simulink model "afe_dq_ttype"  (R2026b)
settings: Solver=ode23tb  StopTime=param.sim.simlength  FixedStep=param.sim.tc  MaxStep=param.glb_time.tc
values from neighbouring files (symbols this model uses):
  param = struct()    [init_model.m]
undefined symbols (not defined in the file or in its folder): magnitude
libraries: fl_lib x281, nesl_utility x136, igbt_simple_2th_lib x12, single_phase_transformer_lib x3, discrete_time_low_pass_filter x1, threephase_inductor_lib x1, dclink_for_three_levels x1, three_phase_three_level_ttype_inverter_ideal_switch_based_model x1, three_phase_three_levels_PWM_modulator x1, three_phase_bridge_three_level_ttype_igbt_simple_2th x1, three_phase_voltage_with_frt_emulator_mfcn x1
(part 3 of 8)

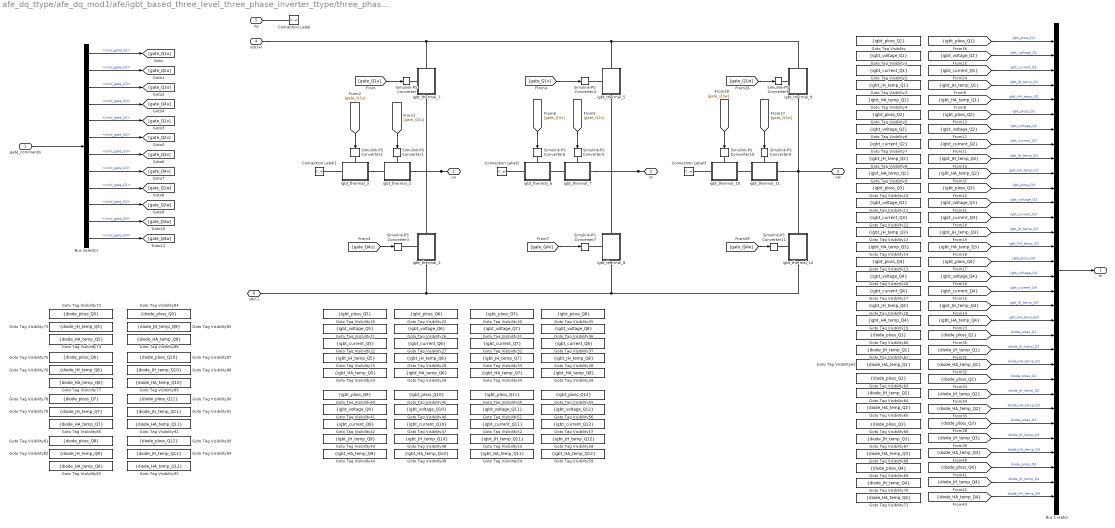
== system afe_dq_ttype/afe_dq_mod1/afe/igbt_based_three_level_three_phase_inverter_ttype/three_phase_inverter_igbt_2th_based_ttype ==
  gate_commands : Inport
  Bus Creator : BusCreator  Inputs=32
  Bus Selector : BusSelector  OutputSignals=gate_cmds_phu.cmd_gate_Q1,gate_cmds_phu.cmd_gate_Q2,gate_cmds_phu.cmd_gate_Q3,gate_cmds_phu.cmd_gate_Q4,gate_cmds_phv.cmd_gate_Q1,gate_cmds_phv.cmd_gate_Q2,gate_cmds_phv.cmd_gate_Q3,gate_cmds_phv.cmd_gate_Q4,gate_cmds_phw.cmd_gate_Q1,gate_cmds_phw.cmd_gate_Q2,gate_cmds_phw.cmd_gate_Q3,gate_cmds_phw.cmd_gate_Q4
  Connection Label{,1..3} (4 alike) : ConnectionLabel  Label=np
  Goto Tag Visibility : GotoTagVisibility  GotoTag=igbt_ploss_Q1
  Goto Tag Visibility1 : GotoTagVisibility  GotoTag=igbt_voltage_Q1
  Goto Tag Visibility10 : GotoTagVisibility  GotoTag=igbt_ploss_Q3
  Goto Tag Visibility11 : GotoTagVisibility  GotoTag=igbt_voltage_Q3
  Goto Tag Visibility12 : GotoTagVisibility  GotoTag=igbt_current_Q3
  Goto Tag Visibility13 : GotoTagVisibility  GotoTag=igbt_JH_temp_Q3
  Goto Tag Visibility14 : GotoTagVisibility  GotoTag=igbt_HA_temp_Q3
  Goto Tag Visibility15 : GotoTagVisibility  GotoTag=igbt_ploss_Q4
  Goto Tag Visibility16 : GotoTagVisibility  GotoTag=igbt_voltage_Q4
  Goto Tag Visibility17 : GotoTagVisibility  GotoTag=igbt_current_Q4
  Goto Tag Visibility18 : GotoTagVisibility  GotoTag=igbt_JH_temp_Q4
  Goto Tag Visibility19 : GotoTagVisibility  GotoTag=igbt_HA_temp_Q4
  Goto Tag Visibility2 : GotoTagVisibility  GotoTag=igbt_current_Q1
  Goto Tag Visibility20 : GotoTagVisibility  GotoTag=igbt_ploss_Q5
  Goto Tag Visibility21 : GotoTagVisibility  GotoTag=igbt_voltage_Q5
  Goto Tag Visibility22 : GotoTagVisibility  GotoTag=igbt_current_Q5
  Goto Tag Visibility23 : GotoTagVisibility  GotoTag=igbt_JH_temp_Q5
  Goto Tag Visibility24 : GotoTagVisibility  GotoTag=igbt_HA_temp_Q5
  Goto Tag Visibility25 : GotoTagVisibility  GotoTag=igbt_ploss_Q6
  Goto Tag Visibility26 : GotoTagVisibility  GotoTag=igbt_voltage_Q6
  Goto Tag Visibility27 : GotoTagVisibility  GotoTag=igbt_current_Q6
  Goto Tag Visibility28 : GotoTagVisibility  GotoTag=igbt_JH_temp_Q6
  Goto Tag Visibility29 : GotoTagVisibility  GotoTag=igbt_HA_temp_Q6
  Goto Tag Visibility3 : GotoTagVisibility  GotoTag=igbt_JH_temp_Q1
  Goto Tag Visibility30 : GotoTagVisibility  GotoTag=igbt_ploss_Q7
  Goto Tag Visibility31 : GotoTagVisibility  GotoTag=igbt_voltage_Q7
  Goto Tag Visibility32 : GotoTagVisibility  GotoTag=igbt_current_Q7
  Goto Tag Visibility33 : GotoTagVisibility  GotoTag=igbt_JH_temp_Q7
  Goto Tag Visibility34 : GotoTagVisibility  GotoTag=igbt_HA_temp_Q7
  Goto Tag Visibility35 : GotoTagVisibility  GotoTag=igbt_ploss_Q8
  Goto Tag Visibility36 : GotoTagVisibility  GotoTag=igbt_voltage_Q8
  Goto Tag Visibility37 : GotoTagVisibility  GotoTag=igbt_current_Q8
  Goto Tag Visibility38 : GotoTagVisibility  GotoTag=igbt_JH_temp_Q8
  Goto Tag Visibility39 : GotoTagVisibility  GotoTag=igbt_HA_temp_Q8
  Goto Tag Visibility4 : GotoTagVisibility  GotoTag=igbt_HA_temp_Q1
  Goto Tag Visibility40 : GotoTagVisibility  GotoTag=igbt_ploss_Q9
  Goto Tag Visibility41 : GotoTagVisibility  GotoTag=igbt_voltage_Q9
  Goto Tag Visibility42 : GotoTagVisibility  GotoTag=igbt_current_Q9
  Goto Tag Visibility43 : GotoTagVisibility  GotoTag=igbt_JH_temp_Q9
  Goto Tag Visibility44 : GotoTagVisibility  GotoTag=igbt_HA_temp_Q9
  Goto Tag Visibility45 : GotoTagVisibility  GotoTag=igbt_ploss_Q10
  Goto Tag Visibility46 : GotoTagVisibility  GotoTag=igbt_voltage_Q10
  Goto Tag Visibility47 : GotoTagVisibility  GotoTag=igbt_current_Q10
  Goto Tag Visibility48 : GotoTagVisibility  GotoTag=igbt_JH_temp_Q10
  Goto Tag Visibility49 : GotoTagVisibility  GotoTag=igbt_HA_temp_Q10
  Goto Tag Visibility5 : GotoTagVisibility  GotoTag=igbt_ploss_Q2
  Goto Tag Visibility50 : GotoTagVisibility  GotoTag=igbt_ploss_Q11
  Goto Tag Visibility51 : GotoTagVisibility  GotoTag=igbt_voltage_Q11
  Goto Tag Visibility52 : GotoTagVisibility  GotoTag=igbt_current_Q11
  Goto Tag Visibility53 : GotoTagVisibility  GotoTag=igbt_JH_temp_Q11
  Goto Tag Visibility54 : GotoTagVisibility  GotoTag=igbt_HA_temp_Q11
  Goto Tag Visibility55 : GotoTagVisibility  GotoTag=igbt_ploss_Q12
  Goto Tag Visibility56 : GotoTagVisibility  GotoTag=igbt_voltage_Q12
  Goto Tag Visibility57 : GotoTagVisibility  GotoTag=igbt_current_Q12
  Goto Tag Visibility58 : GotoTagVisibility  GotoTag=igbt_JH_temp_Q12
  Goto Tag Visibility59 : GotoTagVisibility  GotoTag=igbt_HA_temp_Q12
  Goto Tag Visibility6 : GotoTagVisibility  GotoTag=igbt_voltage_Q2
  Goto Tag Visibility60 : GotoTagVisibility  GotoTag=diode_ploss_Q1
  Goto Tag Visibility61 : GotoTagVisibility  GotoTag=diode_JH_temp_Q1
  Goto Tag Visibility62 : GotoTagVisibility  GotoTag=diode_HA_temp_Q1
  Goto Tag Visibility63 : GotoTagVisibility  GotoTag=diode_ploss_Q2
  Goto Tag Visibility64 : GotoTagVisibility  GotoTag=diode_JH_temp_Q2
  Goto Tag Visibility65 : GotoTagVisibility  GotoTag=diode_HA_temp_Q2
  Goto Tag Visibility66 : GotoTagVisibility  GotoTag=diode_ploss_Q3
  Goto Tag Visibility67 : GotoTagVisibility  GotoTag=diode_JH_temp_Q3
  Goto Tag Visibility68 : GotoTagVisibility  GotoTag=diode_HA_temp_Q3
  Goto Tag Visibility69 : GotoTagVisibility  GotoTag=diode_ploss_Q4
  Goto Tag Visibility7 : GotoTagVisibility  GotoTag=igbt_current_Q2
  Goto Tag Visibility70 : GotoTagVisibility  GotoTag=diode_JH_temp_Q4
  Goto Tag Visibility71 : GotoTagVisibility  GotoTag=diode_HA_temp_Q4
  Goto Tag Visibility72 : GotoTagVisibility  GotoTag=diode_ploss_Q5
  Goto Tag Visibility73 : GotoTagVisibility  GotoTag=diode_JH_temp_Q5
  Goto Tag Visibility74 : GotoTagVisibility  GotoTag=diode_HA_temp_Q5
  Goto Tag Visibility75 : GotoTagVisibility  GotoTag=diode_ploss_Q6
  Goto Tag Visibility76 : GotoTagVisibility  GotoTag=diode_JH_temp_Q6
  Goto Tag Visibility77 : GotoTagVisibility  GotoTag=diode_HA_temp_Q6
  Goto Tag Visibility78 : GotoTagVisibility  GotoTag=diode_ploss_Q7
  Goto Tag Visibility79 : GotoTagVisibility  GotoTag=diode_JH_temp_Q7
  Goto Tag Visibility8 : GotoTagVisibility  GotoTag=igbt_JH_temp_Q2
  Goto Tag Visibility80 : GotoTagVisibility  GotoTag=diode_HA_temp_Q7
  Goto Tag Visibility81 : GotoTagVisibility  GotoTag=diode_ploss_Q8
  Goto Tag Visibility82 : GotoTagVisibility  GotoTag=diode_JH_temp_Q8
  Goto Tag Visibility83 : GotoTagVisibility  GotoTag=diode_HA_temp_Q8
  Goto Tag Visibility84 : GotoTagVisibility  GotoTag=diode_ploss_Q9
  Goto Tag Visibility85 : GotoTagVisibility  GotoTag=diode_JH_temp_Q9
  Goto Tag Visibility86 : GotoTagVisibility  GotoTag=diode_HA_temp_Q9
  Goto Tag Visibility87 : GotoTagVisibility  GotoTag=diode_ploss_Q10
  Goto Tag Visibility88 : GotoTagVisibility  GotoTag=diode_JH_temp_Q10
  Goto Tag Visibility89 : GotoTagVisibility  GotoTag=diode_HA_temp_Q10
  Goto Tag Visibility9 : GotoTagVisibility  GotoTag=igbt_HA_temp_Q2
  Goto Tag Visibility90 : GotoTagVisibility  GotoTag=diode_ploss_Q11
  Goto Tag Visibility91 : GotoTagVisibility  GotoTag=diode_JH_temp_Q11
  Goto Tag Visibility92 : GotoTagVisibility  GotoTag=diode_HA_temp_Q11
  Goto Tag Visibility93 : GotoTagVisibility  GotoTag=diode_ploss_Q12
  Goto Tag Visibility94 : GotoTagVisibility  GotoTag=diode_JH_temp_Q12
  Goto Tag Visibility95 : GotoTagVisibility  GotoTag=diode_HA_temp_Q12
  Simulink-PS Converter{,1..11} (12 alike) : nesl_utility/Simulink-PS Converter  PhysicalDomain=network_engine_domain  SubClassName=ps_input  LeftPortType=input  RightPortType=output  PseudoPeriodic=off  Frequencies=[]  NoiseDistribution=none  NoiseParameters=[]  Unit=1  AffineConversion=on  FilteringAndDerivatives=provide  SimscapeFilterOrder=1  InputFilterTimeConstant=0.001  UdotUserProvided=0
  igbt_thermal_1 : Subsystem
      settings: PortSchema="{\"entries\":[{\"content\":{\"sides\":[{\"content\":{\"connectorIds\":[\"LConn1\"]},\"type\":\"ConnectorPlacement.EquallySpacedRectSide\",\"uuid\":\"9277da8d-d460-43e6-8478-dd662f15d226\"},{\"content\":{\"connectorIds\":[],\"side\":\"RIGHT\"},\"type\":\"ConnectorPlacement.EquallySpacedRectSide\",\"uuid\":\"a7ece396-f1d9-4f4f-a05b-db1fc65d6e1d\"},{\"content\":{\"connectorIds\":[\"LConn2\"],\"side\":\"TOP\"},\"type\":\"ConnectorPlacement.EquallySpacedRectSide\",\"uuid\":\"fdd70777-e9cf-4317-afb6-cae87f75d5b0\"},{\"content\":{\"connectorIds\":[\"RConn1\"],\"side\":\"BOTTOM\"},\"type\":\"ConnectorPlacement.EquallySpacedRectSide\",\"uuid\":\"2353ed68-b1a1-4775-9ca9-31e268d5443b\"}]},\"type\":\"ConnectorPlacement.EquallySpacedConnector\",\"uuid\":\"d5479f4c-4e65-4791-adcb-73df11f88590\"}],\"packageUris\":[\"http://schema.mathworks.com/mf0/Connector/R2020b\"],\"version\":\"1.0\"}"
  igbt_thermal_10 : Subsystem
      settings: PortSchema="{\"entries\":[{\"content\":{\"sides\":[{\"content\":{\"connectorIds\":[\"LConn1\"]},\"type\":\"ConnectorPlacement.EquallySpacedRectSide\",\"uuid\":\"9277da8d-d460-43e6-8478-dd662f15d226\"},{\"content\":{\"connectorIds\":[],\"side\":\"RIGHT\"},\"type\":\"ConnectorPlacement.EquallySpacedRectSide\",\"uuid\":\"a7ece396-f1d9-4f4f-a05b-db1fc65d6e1d\"},{\"content\":{\"connectorIds\":[\"LConn2\"],\"side\":\"TOP\"},\"type\":\"ConnectorPlacement.EquallySpacedRectSide\",\"uuid\":\"fdd70777-e9cf-4317-afb6-cae87f75d5b0\"},{\"content\":{\"connectorIds\":[\"RConn1\"],\"side\":\"BOTTOM\"},\"type\":\"ConnectorPlacement.EquallySpacedRectSide\",\"uuid\":\"2353ed68-b1a1-4775-9ca9-31e268d5443b\"}]},\"type\":\"ConnectorPlacement.EquallySpacedConnector\",\"uuid\":\"d5479f4c-4e65-4791-adcb-73df11f88590\"}],\"packageUris\":[\"http://schema.mathworks.com/mf0/Connector/R2020b\"],\"version\":\"1.0\"}"
  igbt_thermal_11 : Subsystem
      settings: PortSchema="{\"entries\":[{\"content\":{\"sides\":[{\"content\":{\"connectorIds\":[\"LConn1\"]},\"type\":\"ConnectorPlacement.EquallySpacedRectSide\",\"uuid\":\"9277da8d-d460-43e6-8478-dd662f15d226\"},{\"content\":{\"connectorIds\":[],\"side\":\"RIGHT\"},\"type\":\"ConnectorPlacement.EquallySpacedRectSide\",\"uuid\":\"a7ece396-f1d9-4f4f-a05b-db1fc65d6e1d\"},{\"content\":{\"connectorIds\":[\"LConn2\"],\"side\":\"TOP\"},\"type\":\"ConnectorPlacement.EquallySpacedRectSide\",\"uuid\":\"fdd70777-e9cf-4317-afb6-cae87f75d5b0\"},{\"content\":{\"connectorIds\":[\"RConn1\"],\"side\":\"BOTTOM\"},\"type\":\"ConnectorPlacement.EquallySpacedRectSide\",\"uuid\":\"2353ed68-b1a1-4775-9ca9-31e268d5443b\"}]},\"type\":\"ConnectorPlacement.EquallySpacedConnector\",\"uuid\":\"d5479f4c-4e65-4791-adcb-73df11f88590\"}],\"packageUris\":[\"http://schema.mathworks.com/mf0/Connector/R2020b\"],\"version\":\"1.0\"}"
  igbt_thermal_12 : Subsystem
      settings: PortSchema="{\"entries\":[{\"content\":{\"sides\":[{\"content\":{\"connectorIds\":[\"LConn1\"]},\"type\":\"ConnectorPlacement.EquallySpacedRectSide\",\"uuid\":\"9277da8d-d460-43e6-8478-dd662f15d226\"},{\"content\":{\"connectorIds\":[],\"side\":\"RIGHT\"},\"type\":\"ConnectorPlacement.EquallySpacedRectSide\",\"uuid\":\"a7ece396-f1d9-4f4f-a05b-db1fc65d6e1d\"},{\"content\":{\"connectorIds\":[\"LConn2\"],\"side\":\"TOP\"},\"type\":\"ConnectorPlacement.EquallySpacedRectSide\",\"uuid\":\"fdd70777-e9cf-4317-afb6-cae87f75d5b0\"},{\"content\":{\"connectorIds\":[\"RConn1\"],\"side\":\"BOTTOM\"},\"type\":\"ConnectorPlacement.EquallySpacedRectSide\",\"uuid\":\"2353ed68-b1a1-4775-9ca9-31e268d5443b\"}]},\"type\":\"ConnectorPlacement.EquallySpacedConnector\",\"uuid\":\"d5479f4c-4e65-4791-adcb-73df11f88590\"}],\"packageUris\":[\"http://schema.mathworks.com/mf0/Connector/R2020b\"],\"version\":\"1.0\"}"
  igbt_thermal_2 : Subsystem
      settings: PortSchema="{\"entries\":[{\"content\":{\"sides\":[{\"content\":{\"connectorIds\":[\"LConn1\"]},\"type\":\"ConnectorPlacement.EquallySpacedRectSide\",\"uuid\":\"9277da8d-d460-43e6-8478-dd662f15d226\"},{\"content\":{\"connectorIds\":[],\"side\":\"RIGHT\"},\"type\":\"ConnectorPlacement.EquallySpacedRectSide\",\"uuid\":\"a7ece396-f1d9-4f4f-a05b-db1fc65d6e1d\"},{\"content\":{\"connectorIds\":[\"LConn2\"],\"side\":\"TOP\"},\"type\":\"ConnectorPlacement.EquallySpacedRectSide\",\"uuid\":\"fdd70777-e9cf-4317-afb6-cae87f75d5b0\"},{\"content\":{\"connectorIds\":[\"RConn1\"],\"side\":\"BOTTOM\"},\"type\":\"ConnectorPlacement.EquallySpacedRectSide\",\"uuid\":\"2353ed68-b1a1-4775-9ca9-31e268d5443b\"}]},\"type\":\"ConnectorPlacement.EquallySpacedConnector\",\"uuid\":\"d5479f4c-4e65-4791-adcb-73df11f88590\"}],\"packageUris\":[\"http://schema.mathworks.com/mf0/Connector/R2020b\"],\"version\":\"1.0\"}"
  igbt_thermal_3 : Subsystem
      settings: PortSchema="{\"entries\":[{\"content\":{\"sides\":[{\"content\":{\"connectorIds\":[\"LConn1\"]},\"type\":\"ConnectorPlacement.EquallySpacedRectSide\",\"uuid\":\"9277da8d-d460-43e6-8478-dd662f15d226\"},{\"content\":{\"side\":\"RIGHT\"},\"type\":\"ConnectorPlacement.EquallySpacedRectSide\",\"uuid\":\"a7ece396-f1d9-4f4f-a05b-db1fc65d6e1d\"},{\"content\":{\"connectorIds\":[\"LConn2\"],\"side\":\"TOP\"},\"type\":\"ConnectorPlacement.EquallySpacedRectSide\",\"uuid\":\"fdd70777-e9cf-4317-afb6-cae87f75d5b0\"},{\"content\":{\"connectorIds\":[\"RConn1\"],\"side\":\"BOTTOM\"},\"type\":\"ConnectorPlacement.EquallySpacedRectSide\",\"uuid\":\"2353ed68-b1a1-4775-9ca9-31e268d5443b\"}]},\"type\":\"ConnectorPlacement.EquallySpacedConnector\",\"uuid\":\"d5479f4c-4e65-4791-adcb-73df11f88590\"}],\"packageUris\":[\"http://schema.mathworks.com/mf0/Connector/R2020b\"],\"version\":\"1.0\"}"
  igbt_thermal_4 : Subsystem
      settings: PortSchema="{\"entries\":[{\"content\":{\"sides\":[{\"content\":{\"connectorIds\":[\"LConn1\"]},\"type\":\"ConnectorPlacement.EquallySpacedRectSide\",\"uuid\":\"9277da8d-d460-43e6-8478-dd662f15d226\"},{\"content\":{\"connectorIds\":[],\"side\":\"RIGHT\"},\"type\":\"ConnectorPlacement.EquallySpacedRectSide\",\"uuid\":\"a7ece396-f1d9-4f4f-a05b-db1fc65d6e1d\"},{\"content\":{\"connectorIds\":[\"LConn2\"],\"side\":\"TOP\"},\"type\":\"ConnectorPlacement.EquallySpacedRectSide\",\"uuid\":\"fdd70777-e9cf-4317-afb6-cae87f75d5b0\"},{\"content\":{\"connectorIds\":[\"RConn1\"],\"side\":\"BOTTOM\"},\"type\":\"ConnectorPlacement.EquallySpacedRectSide\",\"uuid\":\"2353ed68-b1a1-4775-9ca9-31e268d5443b\"}]},\"type\":\"ConnectorPlacement.EquallySpacedConnector\",\"uuid\":\"d5479f4c-4e65-4791-adcb-73df11f88590\"}],\"packageUris\":[\"http://schema.mathworks.com/mf0/Connector/R2020b\"],\"version\":\"1.0\"}"
  igbt_thermal_5 : Subsystem
      settings: PortSchema="{\"entries\":[{\"content\":{\"sides\":[{\"content\":{\"connectorIds\":[\"LConn1\"]},\"type\":\"ConnectorPlacement.EquallySpacedRectSide\",\"uuid\":\"9277da8d-d460-43e6-8478-dd662f15d226\"},{\"content\":{\"connectorIds\":[],\"side\":\"RIGHT\"},\"type\":\"ConnectorPlacement.EquallySpacedRectSide\",\"uuid\":\"a7ece396-f1d9-4f4f-a05b-db1fc65d6e1d\"},{\"content\":{\"connectorIds\":[\"LConn2\"],\"side\":\"TOP\"},\"type\":\"ConnectorPlacement.EquallySpacedRectSide\",\"uuid\":\"fdd70777-e9cf-4317-afb6-cae87f75d5b0\"},{\"content\":{\"connectorIds\":[\"RConn1\"],\"side\":\"BOTTOM\"},\"type\":\"ConnectorPlacement.EquallySpacedRectSide\",\"uuid\":\"2353ed68-b1a1-4775-9ca9-31e268d5443b\"}]},\"type\":\"ConnectorPlacement.EquallySpacedConnector\",\"uuid\":\"d5479f4c-4e65-4791-adcb-73df11f88590\"}],\"packageUris\":[\"http://schema.mathworks.com/mf0/Connector/R2020b\"],\"version\":\"1.0\"}"
  igbt_thermal_6 : Subsystem
      settings: PortSchema="{\"entries\":[{\"content\":{\"sides\":[{\"content\":{\"connectorIds\":[\"LConn1\"]},\"type\":\"ConnectorPlacement.EquallySpacedRectSide\",\"uuid\":\"9277da8d-d460-43e6-8478-dd662f15d226\"},{\"content\":{\"side\":\"RIGHT\"},\"type\":\"ConnectorPlacement.EquallySpacedRectSide\",\"uuid\":\"a7ece396-f1d9-4f4f-a05b-db1fc65d6e1d\"},{\"content\":{\"connectorIds\":[\"LConn2\"],\"side\":\"TOP\"},\"type\":\"ConnectorPlacement.EquallySpacedRectSide\",\"uuid\":\"fdd70777-e9cf-4317-afb6-cae87f75d5b0\"},{\"content\":{\"connectorIds\":[\"RConn1\"],\"side\":\"BOTTOM\"},\"type\":\"ConnectorPlacement.EquallySpacedRectSide\",\"uuid\":\"2353ed68-b1a1-4775-9ca9-31e268d5443b\"}]},\"type\":\"ConnectorPlacement.EquallySpacedConnector\",\"uuid\":\"d5479f4c-4e65-4791-adcb-73df11f88590\"}],\"packageUris\":[\"http://schema.mathworks.com/mf0/Connector/R2020b\"],\"version\":\"1.0\"}"
  igbt_thermal_7 : Subsystem
      settings: PortSchema="{\"entries\":[{\"content\":{\"sides\":[{\"content\":{\"connectorIds\":[\"LConn1\"]},\"type\":\"ConnectorPlacement.EquallySpacedRectSide\",\"uuid\":\"9277da8d-d460-43e6-8478-dd662f15d226\"},{\"content\":{\"connectorIds\":[],\"side\":\"RIGHT\"},\"type\":\"ConnectorPlacement.EquallySpacedRectSide\",\"uuid\":\"a7ece396-f1d9-4f4f-a05b-db1fc65d6e1d\"},{\"content\":{\"connectorIds\":[\"LConn2\"],\"side\":\"TOP\"},\"type\":\"ConnectorPlacement.EquallySpacedRectSide\",\"uuid\":\"fdd70777-e9cf-4317-afb6-cae87f75d5b0\"},{\"content\":{\"connectorIds\":[\"RConn1\"],\"side\":\"BOTTOM\"},\"type\":\"ConnectorPlacement.EquallySpacedRectSide\",\"uuid\":\"2353ed68-b1a1-4775-9ca9-31e268d5443b\"}]},\"type\":\"ConnectorPlacement.EquallySpacedConnector\",\"uuid\":\"d5479f4c-4e65-4791-adcb-73df11f88590\"}],\"packageUris\":[\"http://schema.mathworks.com/mf0/Connector/R2020b\"],\"version\":\"1.0\"}"
  igbt_thermal_8 : Subsystem
      settings: PortSchema="{\"entries\":[{\"content\":{\"sides\":[{\"content\":{\"connectorIds\":[\"LConn1\"]},\"type\":\"ConnectorPlacement.EquallySpacedRectSide\",\"uuid\":\"9277da8d-d460-43e6-8478-dd662f15d226\"},{\"content\":{\"connectorIds\":[],\"side\":\"RIGHT\"},\"type\":\"ConnectorPlacement.EquallySpacedRectSide\",\"uuid\":\"a7ece396-f1d9-4f4f-a05b-db1fc65d6e1d\"},{\"content\":{\"connectorIds\":[\"LConn2\"],\"side\":\"TOP\"},\"type\":\"ConnectorPlacement.EquallySpacedRectSide\",\"uuid\":\"fdd70777-e9cf-4317-afb6-cae87f75d5b0\"},{\"content\":{\"connectorIds\":[\"RConn1\"],\"side\":\"BOTTOM\"},\"type\":\"ConnectorPlacement.EquallySpacedRectSide\",\"uuid\":\"2353ed68-b1a1-4775-9ca9-31e268d5443b\"}]},\"type\":\"ConnectorPlacement.EquallySpacedConnector\",\"uuid\":\"d5479f4c-4e65-4791-adcb-73df11f88590\"}],\"packageUris\":[\"http://schema.mathworks.com/mf0/Connector/R2020b\"],\"version\":\"1.0\"}"
  igbt_thermal_9 : Subsystem
      settings: PortSchema="{\"entries\":[{\"content\":{\"sides\":[{\"content\":{\"connectorIds\":[\"LConn1\"]},\"type\":\"ConnectorPlacement.EquallySpacedRectSide\",\"uuid\":\"9277da8d-d460-43e6-8478-dd662f15d226\"},{\"content\":{\"connectorIds\":[],\"side\":\"RIGHT\"},\"type\":\"ConnectorPlacement.EquallySpacedRectSide\",\"uuid\":\"a7ece396-f1d9-4f4f-a05b-db1fc65d6e1d\"},{\"content\":{\"connectorIds\":[\"LConn2\"],\"side\":\"TOP\"},\"type\":\"ConnectorPlacement.EquallySpacedRectSide\",\"uuid\":\"fdd70777-e9cf-4317-afb6-cae87f75d5b0\"},{\"content\":{\"connectorIds\":[\"RConn1\"],\"side\":\"BOTTOM\"},\"type\":\"ConnectorPlacement.EquallySpacedRectSide\",\"uuid\":\"2353ed68-b1a1-4775-9ca9-31e268d5443b\"}]},\"type\":\"ConnectorPlacement.EquallySpacedConnector\",\"uuid\":\"d5479f4c-4e65-4791-adcb-73df11f88590\"}],\"packageUris\":[\"http://schema.mathworks.com/mf0/Connector/R2020b\"],\"version\":\"1.0\"}"
  uu : PMIOPort  Side=Left
  uv : PMIOPort  Port=2  Side=Left
  uw : PMIOPort  Port=3  Side=Left
  udc(+) : PMIOPort  Port=4  Side=Right
  np : PMIOPort  Port=5  Side=Right
  udc(-) : PMIOPort  Port=6  Side=Right
  m : Outport
  wires:
  [gate_Q4u] -> Simulink-PS Converter3/1
  [gate_Q3u] -> Simulink-PS Converter2/1
  [gate_Q2u] -> Simulink-PS Converter1/1
  [gate_Q1u] -> Simulink-PS Converter/1
  [gate_Q1v] -> Simulink-PS Converter4/1
  [gate_Q2v] -> Simulink-PS Converter5/1
  [gate_Q3v] -> Simulink-PS Converter6/1
  [gate_Q4v] -> Simulink-PS Converter7/1
  gate_commands/1 -> Bus Selector/1
  [igbt_voltage_Q1] -> Bus Creator/2  "igbt_voltage_Q1"
  [igbt_current_Q4] -> Bus Creator/18  "igbt_current_Q4"
  [igbt_voltage_Q2] -> Bus Creator/7  "igbt_voltage_Q2"
  [igbt_ploss_Q2] -> Bus Creator/6  "igbt_ploss_Q2"
  Bus Creator/1 -> m/1
  [igbt_ploss_Q3] -> Bus Creator/11  "igbt_ploss_Q3"
  [igbt_HA_temp_Q1] -> Bus Creator/5  "igbt_HA_temp_Q1"
  [igbt_ploss_Q1] -> Bus Creator/1  "igbt_ploss_Q1"
  [igbt_voltage_Q4] -> Bus Creator/17  "igbt_voltage_Q4"
  [igbt_ploss_Q4] -> Bus Creator/16  "igbt_ploss_Q4"
  [igbt_JH_temp_Q4] -> Bus Creator/19  "igbt_JH_temp_Q4"
  [igbt_voltage_Q3] -> Bus Creator/12  "igbt_voltage_Q3"
  [igbt_current_Q1] -> Bus Creator/3  "igbt_current_Q1"
  [igbt_HA_temp_Q4] -> Bus Creator/20  "igbt_HA_temp_Q4"
  [igbt_JH_temp_Q3] -> Bus Creator/14  "igbt_JH_temp_Q3"
  [igbt_current_Q2] -> Bus Creator/8  "igbt_current_Q2"
  [igbt_HA_temp_Q2] -> Bus Creator/10  "igbt_HA_temp_Q2"
  [igbt_JH_temp_Q2] -> Bus Creator/9  "igbt_JH_temp_Q2"
  [igbt_JH_temp_Q1] -> Bus Creator/4  "igbt_JH_temp_Q1"
  [igbt_current_Q3] -> Bus Creator/13  "igbt_current_Q3"
  [igbt_HA_temp_Q3] -> Bus Creator/15  "igbt_HA_temp_Q3"
  [gate_Q4w] -> Simulink-PS Converter11/1
  [gate_Q3w] -> Simulink-PS Converter10/1
  [gate_Q2w] -> Simulink-PS Converter9/1
  [gate_Q1w] -> Simulink-PS Converter8/1
  [diode_ploss_Q1] -> Bus Creator/21  "diode_ploss_Q1"
  [diode_JH_temp_Q1] -> Bus Creator/22  "diode_JH_temp_Q1"
  [diode_HA_temp_Q1] -> Bus Creator/23  "diode_HA_temp_Q1"
  [diode_ploss_Q2] -> Bus Creator/24  "diode_ploss_Q2"
  [diode_JH_temp_Q2] -> Bus Creator/25  "diode_JH_temp_Q2"
  [diode_HA_temp_Q2] -> Bus Creator/26  "diode_HA_temp_Q2"
  [diode_ploss_Q3] -> Bus Creator/27  "diode_ploss_Q3"
  [diode_JH_temp_Q3] -> Bus Creator/28  "diode_JH_temp_Q3"
  [diode_HA_temp_Q3] -> Bus Creator/29  "diode_HA_temp_Q3"
  [diode_HA_temp_Q4] -> Bus Creator/32  "diode_HA_temp_Q4"
  [diode_JH_temp_Q4] -> Bus Creator/31  "diode_JH_temp_Q4"
  [diode_ploss_Q4] -> Bus Creator/30  "diode_ploss_Q4"
  Bus Selector/1 -> [gate_Q1u]  "<cmd_gate_Q1>"
  Bus Selector/2 -> [gate_Q2u]  "<cmd_gate_Q2>"
  Bus Selector/3 -> [gate_Q3u]  "<cmd_gate_Q3>"
  Bus Selector/9 -> [gate_Q1w]  "<cmd_gate_Q1>"
  Bus Selector/4 -> [gate_Q4u]  "<cmd_gate_Q4>"
  Bus Selector/5 -> [gate_Q1v]  "<cmd_gate_Q1>"
  Bus Selector/6 -> [gate_Q2v]  "<cmd_gate_Q2>"
  Bus Selector/7 -> [gate_Q3v]  "<cmd_gate_Q3>"
  Bus Selector/8 -> [gate_Q4v]  "<cmd_gate_Q4>"
  Bus Selector/10 -> [gate_Q2w]  "<cmd_gate_Q2>"
  Bus Selector/12 -> [gate_Q4w]  "<cmd_gate_Q4>"
  Bus Selector/11 -> [gate_Q3w]  "<cmd_gate_Q3>"
  connections:
  udc(+)/RConn1 -- igbt_thermal_1/LConn2 -- igbt_thermal_5/LConn2 -- igbt_thermal_9/LConn2
  igbt_thermal_4/LConn1 -- Simulink-PS Converter3/RConn1
  igbt_thermal_3/LConn1 -- Simulink-PS Converter2/RConn1
  igbt_thermal_2/LConn1 -- Simulink-PS Converter1/RConn1
  igbt_thermal_1/LConn1 -- Simulink-PS Converter/RConn1
  igbt_thermal_7/LConn1 -- Simulink-PS Converter5/RConn1
  igbt_thermal_6/LConn1 -- Simulink-PS Converter6/RConn1
  igbt_thermal_8/LConn1 -- Simulink-PS Converter7/RConn1
  uu/RConn1 -- igbt_thermal_2/RConn1 -- igbt_thermal_4/LConn2 -- igbt_thermal_1/RConn1
  igbt_thermal_12/RConn1 -- igbt_thermal_8/RConn1 -- udc(-)/RConn1 -- igbt_thermal_4/RConn1
  uv/RConn1 -- igbt_thermal_5/RConn1 -- igbt_thermal_8/LConn2 -- igbt_thermal_7/RConn1
  igbt_thermal_7/LConn2 -- igbt_thermal_6/LConn2
  Connection Label/LConn1 -- np/RConn1
  igbt_thermal_3/RConn1 -- Connection Label1/LConn1
  igbt_thermal_6/RConn1 -- Connection Label2/LConn1
  igbt_thermal_9/RConn1 -- igbt_thermal_12/LConn2 -- igbt_thermal_11/RConn1 -- uw/RConn1
  igbt_thermal_9/LConn1 -- Simulink-PS Converter8/RConn1
  igbt_thermal_3/LConn2 -- igbt_thermal_2/LConn2
  igbt_thermal_12/LConn1 -- Simulink-PS Converter11/RConn1
  igbt_thermal_10/LConn1 -- Simulink-PS Converter10/RConn1
  igbt_thermal_10/RConn1 -- Connection Label3/LConn1
  igbt_thermal_11/LConn1 -- Simulink-PS Converter9/RConn1
  igbt_thermal_11/LConn2 -- igbt_thermal_10/LConn2
  igbt_thermal_5/LConn1 -- Simulink-PS Converter4/RConn1

== system afe_dq_ttype/afe_dq_mod1/afe/sv_pwm/modulator1 ==
  u : Inport
  v : Inport  Port=2
  w : Inport  Port=3
  phase : Inport  Port=4
  Bus Creator : BusCreator  Inputs=3
  three_phase_three_levels_PWM_generator_with_global_TRGO1 : three_phase_three_levels_PWM_modulator/three_phase_three_levels_PWM_generator_with_global_TRGO1  f=param.glb_time.fPWM_AFE  m_up=1  m_low=-1  dead_time=0  pos_cmd_gate=15  neg_cmd_gate=0  polarity=1  tc=param.glb_time.tc  double_sampling=param.glb_time.TRGO_AFE_double_update
      link override gate commands/Bus Selector: OutputSignals=du(t)
      link override gate commands/Bus Selector1: OutputSignals=dv(t)
      link override gate commands/Bus Selector2: OutputSignals=dw(t)
  gate_cmds : Outport
  tag scope: TRGO_afe_module_1=global
  wires:
  [time_afe_module_1] -> three_phase_three_levels_PWM_generator_with_global_TRGO1/1
  Bus Creator/1 -> three_phase_three_levels_PWM_generator_with_global_TRGO1/3
  three_phase_three_levels_PWM_generator_with_global_TRGO1/1 -> [TRGO_afe_module_1]
  u/1 -> Bus Creator/1  "du(t)"
  v/1 -> Bus Creator/2  "dv(t)"
  w/1 -> Bus Creator/3  "dw(t)"
  phase/1 -> three_phase_three_levels_PWM_generator_with_global_TRGO1/2
  three_phase_three_levels_PWM_generator_with_global_TRGO1/2 -> gate_cmds/1

== system afe_dq_ttype/afe_dq_mod1/AFE_control/afe_control/acquisitions/grid_phase_acquisition ==
  grid_phase : Inport
  Quantizer : Quantizer  QuantizationInterval=param.meas.adc_quantization
  Unit Delay : UnitDelay  SampleTime=-1
  Zero-Order Hold : ZeroOrderHold  SampleTime=-1
  grid_phased : Outport
  wires:
  Zero-Order Hold/1 -> Quantizer/1
  Unit Delay/1 -> grid_phased/1
  grid_phase/1 -> Zero-Order Hold/1
  Quantizer/1 -> Unit Delay/1

== system afe_dq_ttype/afe_dq_mod1/AFE_control/afe_control/acquisitions/ig afe quantizzation and one step delay ==
  ig_abc_pu : Inport
  Demux1 : Demux  Outputs=3
  Mux1 : Mux  Inputs=3
  ig afe quantizzation and one step delay : Subsystem
  igd_abc_pu : Outport
  wires:
  Demux1/1 -> ig afe quantizzation and one step delay/1(ig_u_pu)
  Demux1/2 -> ig afe quantizzation and one step delay/2(ig_v_pu)
  ig_abc_pu/1 -> Demux1/1
  Mux1/1 -> igd_abc_pu/1
  Demux1/3 -> ig afe quantizzation and one step delay/3(ig_w_pu)
  ig afe quantizzation and one step delay/2(igd_v_pu) -> Mux1/2
  ig afe quantizzation and one step delay/1(igd_u_pu) -> Mux1/1
  ig afe quantizzation and one step delay/3(igd_w_pu) -> Mux1/3

== system afe_dq_ttype/afe_dq_mod1/AFE_control/afe_control/acquisitions/is afe quantizzation and one step delay ==
  is_abc_pu : Inport
  Demux : Demux  Outputs=3
  Mux : Mux  Inputs=3
  is afe quantizzation and one step delay : Subsystem
  isd_abc_pu : Outport
  wires:
  is afe quantizzation and one step delay/2(isd_v_pu) -> Mux/2
  is_abc_pu/1 -> Demux/1
  is afe quantizzation and one step delay/3(isd_w_pu) -> Mux/3
  is afe quantizzation and one step delay/1(isd_u_pu) -> Mux/1
  Demux/1 -> is afe quantizzation and one step delay/1(is_u_pu)
  Mux/1 -> isd_abc_pu/1
  Demux/3 -> is afe quantizzation and one step delay/3(is_w_pu)
  Demux/2 -> is afe quantizzation and one step delay/2(is_v_pu)

== system afe_dq_ttype/afe_dq_mod1/AFE_control/afe_control/acquisitions/phase_compensation_1 ==
  local_time : Inport
  master_time : Inport  Port=2
  Zero-Order Hold : ZeroOrderHold  SampleTime=-1
  Zero-Order Hold1 : ZeroOrderHold  SampleTime=-1
  alignment_eval_afe1 : Subsystem
  y : Outport
  wires:
  local_time/1 -> Zero-Order Hold/1
  master_time/1 -> Zero-Order Hold1/1
  alignment_eval_afe1/1(dp) -> y/1
  Zero-Order Hold/1 -> alignment_eval_afe1/1(local_time)
  Zero-Order Hold1/1 -> alignment_eval_afe1/2(master_time)

== system afe_dq_ttype/afe_dq_mod1/AFE_control/afe_control/acquisitions/udc_acquisition ==
  udc_pu : Inport
  Quantizer : Quantizer  QuantizationInterval=param.meas.adc_quantization
  Unit Delay : UnitDelay  SampleTime=-1
  Zero-Order Hold : ZeroOrderHold  SampleTime=-1
  udcd_pu : Outport
  wires:
  Quantizer/1 -> Unit Delay/1
  udc_pu/1 -> Zero-Order Hold/1
  Unit Delay/1 -> udcd_pu/1
  Zero-Order Hold/1 -> Quantizer/1

== system afe_dq_ttype/afe_dq_mod1/AFE_control/afe_control/acquisitions/ug afe quantizzation and one step delay ==
  ug_abc_pu : Inport
  Demux : Demux  Outputs=3
  Mux : Mux  Inputs=3
  ug afe quantizzation and one step delay : Subsystem
  ugd_abc_pu : Outport
  wires:
  ug afe quantizzation and one step delay/2(ugd_v_pu) -> Mux/2
  Demux/2 -> ug afe quantizzation and one step delay/2(ug_v_pu)
  Demux/3 -> ug afe quantizzation and one step delay/3(ug_w_pu)
  ug afe quantizzation and one step delay/1(ugd_u_pu) -> Mux/1
  Demux/1 -> ug afe quantizzation and one step delay/1(ug_u_pu)
  ug_abc_pu/1 -> Demux/1
  ug afe quantizzation and one step delay/3(ugd_w_pu) -> Mux/3
  Mux/1 -> ugd_abc_pu/1

== system afe_dq_ttype/afe_dq_mod1/AFE_control/afe_control/current_ctrl/current_transformation ==
  is_a_pu : Inport
  is_b_pu : Inport  Port=2
  is_c_pu : Inport  Port=3
  alphabeta2xieta : MATLAB Function  TreatAsAtomicUnit=on
  uvw2alphabeta : MATLAB Function  TreatAsAtomicUnit=on
  tag scope: id_eta_pu=scoped, id_xi_pu=scoped
  wires:
  is_c_pu/1 -> uvw2alphabeta/3(w)
  alphabeta2xieta/2(eta) -> [id_eta_pu]  "ieta_pu"
  alphabeta2xieta/1(xi) -> [id_xi_pu]  "ixi_pu"
  is_b_pu/1 -> uvw2alphabeta/2(v)
  uvw2alphabeta/2(beta) -> alphabeta2xieta/2(beta)  "ibeta_pu"
  uvw2alphabeta/1(alpha) -> alphabeta2xieta/1(alpha)  "ialpha_pu"
  [phase_grid_pll] -> alphabeta2xieta/3(gamma)
  is_a_pu/1 -> uvw2alphabeta/1(u)

== system afe_dq_ttype/afe_dq_mod1/AFE_control/afe_control/current_ctrl/dq_vector_pi ==
  id : Inport
  id_ref : Inport  Port=2
  iq : Inport  Port=3
  iq_ref : Inport  Port=4
  Sum1 : Sum  Inputs=|-+
  Sum2 : Sum  Inputs=|-+
  bounder1 : Subsystem
  bounder2 : Subsystem
  pi_d : Subsystem
  pi_q : Subsystem
  switch : Subsystem
  vector lenght : Subsystem
  md_sat : Outport
  mq_sat : Outport  Port=2
  wires:
  bounder2/2(clip) -> switch/2(clip 2)
  vector lenght/2(m) -> bounder1/3(m), bounder2/1(m)
  Sum2/1 -> pi_q/1(iq_tilde)
  pi_d/1(ud_out) -> vector lenght/1(md), bounder1/1(md)
  pi_q/1(Vqs_out) -> bounder2/3(mq), vector lenght/2(mq)
  vector lenght/1(m_1) -> bounder1/2(m_1), bounder2/2(m_1)
  switch/1(clip) -> pi_q/2(clip), pi_d/2(clip)
  iq/1 -> Sum2/1
  Sum1/1 -> pi_d/1(id_tilde)
  bounder1/2(clip) -> switch/1(clip 1)
  id/1 -> Sum1/1
  bounder1/1(md_sat) -> md_sat/1
  bounder2/1(mq_sat) -> mq_sat/1
  id_ref/1 -> Sum1/2
  iq_ref/1 -> Sum2/2

== system afe_dq_ttype/afe_dq_mod1/AFE_control/afe_control/current_ctrl/zero_current_ctrl ==
  ualpha_ctrl_afe : Inport
  ubeta_ctrl_afe : Inport  Port=2
  Bus Creator1 : BusCreator  Inputs=3
  iz : Subsystem
  zero_sequence_current_ctrl : Subsystem
  uabg_ctrl_out : Outport
  wires:
  Bus Creator1/1 -> uabg_ctrl_out/1
  ualpha_ctrl_afe/1 -> Bus Creator1/1  "ualpha_ctrl_afe"
  ubeta_ctrl_afe/1 -> Bus Creator1/2  "ubeta_ctrl_afe"
  iz/1(iz) -> zero_sequence_current_ctrl/1(iz)
  zero_sequence_current_ctrl/1(ugamma_afe) -> Bus Creator1/3  "ugamma_ctrl_afe"

== system afe_dq_ttype/afe_dq_mod1/AFE_control/afe_control/data_to_worspace_module_1/dq_pll ==
  Bus Creator1 : BusCreator  Inputs=8
  dqPLLs : Outport
  wires:
  [phase_grid_fht_simulink_pll] -> Bus Creator1/5  "phase_grid_fht_simulink_pll"
  [omega_grid_fht_simulink_pll] -> Bus Creator1/6  "omega_grid_fht_simulink_pll"
  [omega_grid_fhtsr_dqpll] -> Bus Creator1/8  "omega_grid_fhtsr_dqpll"
  [phase_grid_fhtsr_dqpll] -> Bus Creator1/7  "phase_grid_fhtsr_dqpll"
  [omega_grid_dqpll_ccaller] -> Bus Creator1/4  "omega_grid_dqpll_ccaller"
  [phase_grid_dqpll_ccaller] -> Bus Creator1/3  "phase_grid_dqpll_ccaller"
  [omega_grid_pu_dqpll] -> Bus Creator1/2  "omega_grid_pu_dqpll"
  [phase_grid_dqpll] -> Bus Creator1/1  "phase_grid_dqpll"
  Bus Creator1/1 -> dqPLLs/1

== system afe_dq_ttype/afe_dq_mod1/AFE_control/afe_control/data_to_worspace_module_1/pwr_meter ==
  Bus Creator1 : BusCreator  Inputs=4
  m_pwr_meter : Outport
  wires:
  [u_grid_pu_rms] -> Bus Creator1/2  "u_grid_pu_rms"
  Bus Creator1/1 -> m_pwr_meter/1
  [pwr_act_grid] -> Bus Creator1/3  "pwr_act_grid"
  [pwr_react_grid] -> Bus Creator1/4  "pwr_react_grid"
  [i_grid_pu_rms] -> Bus Creator1/1  "i_grid_pu_rms"

== system afe_dq_ttype/afe_dq_mod1/AFE_control/afe_control/grid_voltage_phase_lock_loops/FHT-PLL ==
  ug_abc_pu : Inport
  pll_stageA : Subsystem
  pll_stageB : Subsystem
  gamma_grid_fht_pll : Outport
  omega_grid_fht_pll : Outport  Port=2
  wires:
  ug_abc_pu/1 -> pll_stageA/2(ug_abc_pu)
  pll_stageB/2(omega_grid_ddsrf_pll) -> omega_grid_fht_pll/1
  pll_stageA/1(u_grid_xi) -> pll_stageB/1(u_grid_pos_xi)  "u_grid_pos_xi"
  pll_stageA/2(u_grid_eta) -> pll_stageB/2(u_grid_pos_eta)  "u_grid_pos_eta"
  pll_stageB/1(gamma_grid_ddsrf_pll) -> gamma_grid_fht_pll/1, pll_stageA/1(gamma_grid)

== system afe_dq_ttype/afe_dq_mod1/AFE_control/afe_control/grid_voltage_phase_lock_loops/FHT-PLL_simulink ==
  ug_abc_pu : Inport
  pll_stageA : Subsystem
  pll_stageB : Subsystem
  gamma_grid_fht_pll : Outport
  omega_grid_fht_pll : Outport  Port=2
  wires:
  pll_stageB/1(gamma_grid_ddsrf_pll) -> pll_stageA/1(gamma_grid), gamma_grid_fht_pll/1
  pll_stageA/2(u_grid_eta) -> pll_stageB/2(u_grid_pos_eta)  "u_grid_pos_eta"
  pll_stageA/1(u_grid_xi) -> pll_stageB/1(u_grid_pos_xi)  "u_grid_pos_xi"
  pll_stageB/2(omega_grid_ddsrf_pll) -> omega_grid_fht_pll/1
  ug_abc_pu/1 -> pll_stageA/2(ug_abc_pu)

== system afe_dq_ttype/afe_dq_mod1/AFE_control/afe_control/grid_voltage_phase_lock_loops/dq_pll ==
  ug_abc_pu : Inport
  Goto Tag Visibility29 : GotoTagVisibility  GotoTag=Vgrid_unorm_dqpll
  pll_stageA : Subsystem
  pll_stageB : Subsystem
  phase_grid_dqpll : Outport
  omega_grid_pu_dqpll : Outport  Port=2
  wires:
  pll_stageA/2(u_grid_pos_eta) -> pll_stageB/2(u_grid_pos_eta)  "u_grid_pos_eta"
  pll_stageB/1(phase_grid_pll) -> phase_grid_dqpll/1, pll_stageA/1(phase_grid)
  pll_stageA/1(u_grid_pos_xi) -> pll_stageB/1(u_grid_pos_xi)  "u_grid_pos_xi"
  pll_stageB/2(omega_grid_pu_pll) -> omega_grid_pu_dqpll/1
  ug_abc_pu/1 -> pll_stageA/2(ug_abc)

== system afe_dq_ttype/afe_dq_mod1/AFE_control/afe_control/grid_voltage_phase_lock_loops/dq_pll_ccaller ==
  ug_abc_pu : Inport
  Bus Selector : BusSelector  OutputSignals=omega_pu_hat,gamma_hat,u_grid_xi,u_grid_eta,dqpll_pll_state
  C Caller : CCaller  FunctionName=dqpll_grid_process_simulink  PortSpecificationStruct="%)30     .    N H   8    (     @         %    \"     8    !     0         %  0 \"0    $    _    07)G3F%M90  4&]R=$YA;64 4V-O<&4     26YD97@     5'EP90      4VEZ90      27-';&]B86P   X    P    !@    @    $          4    (     0    ,    !         !   P!O=70 #@   #     &    \"     0         !0    @    !     P    $         $  # &]U=  .    .     8    (    !          %    \"     $    &     0         0   ...(+3319 chars)"
  Constant : Constant  Value=param.glb_time.ts_afe
  Data Type Conversion{1..2,4..5} (4 alike) : DataTypeConversion  OutDataTypeStr=single  SaturateOnIntegerOverflow=off  RndMeth=Floor
  Data Type Conversion{6..10} (5 alike) : DataTypeConversion  OutDataTypeStr=double  SaturateOnIntegerOverflow=off  RndMeth=Floor
  Data Type Conversion3 : DataTypeConversion  OutDataTypeStr=uint8  SaturateOnIntegerOverflow=off  RndMeth=Floor
  Demux : Demux  Outputs=3
  Step : Step  Time=0.01  InitialValue=1  FinalValue=0
  first_harmonic_tracker : Scope  NumInputPorts=3
      settings: ActiveDisplayYMinimum=-1.7184470891952515  ActiveDisplayYMaximum=1.8384636640548706
  first_harmonic_tracker_phase_u : Subsystem
  first_harmonic_tracker_phase_v : Subsystem
  first_harmonic_tracker_phase_w : Subsystem
  gamma_hat : Outport  VectorParamsAs1DForOutWhenUnconnected=off
  omega_pu_hat : Outport  Port=2  VectorParamsAs1DForOutWhenUnconnected=off
  dqpll_uxi : Outport  Port=3  VectorParamsAs1DForOutWhenUnconnected=off
  dqpll_ueta : Outport  Port=4  VectorParamsAs1DForOutWhenUnconnected=off
  dqpll_state : Outport  Port=5  VectorParamsAs1DForOutWhenUnconnected=off
  wires:
  Step/1 -> Data Type Conversion3/1
  Constant/1 -> Data Type Conversion1/1
  Data Type Conversion3/1 -> C Caller/1
  Data Type Conversion2/1 -> C Caller/2
  Data Type Conversion4/1 -> C Caller/3
  Data Type Conversion5/1 -> C Caller/4
  Data Type Conversion1/1 -> C Caller/5
  C Caller/1 -> Bus Selector/1
  Bus Selector/1 -> Data Type Conversion6/1  "<omega_pu_hat>"
  Bus Selector/2 -> Data Type Conversion7/1  "<gamma_hat>"
  Bus Selector/3 -> Data Type Conversion8/1  "<u_grid_xi>"
  Bus Selector/4 -> Data Type Conversion9/1  "<u_grid_eta>"
  Bus Selector/5 -> Data Type Conversion10/1  "<dqpll_pll_state>"
  Data Type Conversion7/1 -> gamma_hat/1
  Data Type Conversion10/1 -> dqpll_state/1
  Data Type Conversion8/1 -> dqpll_uxi/1
  Data Type Conversion9/1 -> dqpll_ueta/1
  ug_abc_pu/1 -> Demux/1
  Demux/1 -> first_harmonic_tracker_phase_u/1(u)
  Demux/2 -> first_harmonic_tracker_phase_v/1(u)
  Demux/3 -> first_harmonic_tracker_phase_w/1(u)
  Data Type Conversion6/1 -> omega_pu_hat/1
  first_harmonic_tracker_phase_u/1(u_hat) -> first_harmonic_tracker/1, Data Type Conversion2/1  "tracker_phase_u"
  first_harmonic_tracker_phase_v/1(u_hat) -> first_harmonic_tracker/2, Data Type Conversion4/1  "tracker_phase_v"
  first_harmonic_tracker_phase_w/1(u_hat) -> first_harmonic_tracker/3, Data Type Conversion5/1  "tracker_phase_w"

== system afe_dq_ttype/afe_dq_mod1/AFE_control/afe_control/instantaneus_power/abc2alphabeta ==
  a : Inport
  b : Inport  Port=2
  c : Inport  Port=3
  Gain1 : Gain  Gain=-1/2
  Gain11 : Gain  Gain=-1/2
  Gain2 : Gain  Gain=0
  Gain3 : Gain  Gain=sqrt(3)/2
  Gain4 : Gain  Gain=-sqrt(3)/2
  Gain8 : Gain  Gain=2/3
  Gain9 : Gain  Gain=2/3
  Sum : Sum  Inputs=+++
  Sum1 : Sum  Inputs=+++
  "alpha " : Outport  VectorParamsAs1DForOutWhenUnconnected=off
  "beta " : Outport  Port=2  VectorParamsAs1DForOutWhenUnconnected=off
  wires:
  Gain3/1 -> Sum1/2
  Gain2/1 -> Sum1/1
  Gain11/1 -> Sum/2
  Gain4/1 -> Sum1/3
  Sum1/1 -> Gain9/1
  Gain8/1 -> "alpha "/1
  Sum/1 -> Gain8/1
  c/1 -> Gain4/1, Gain1/1
  Gain9/1 -> "beta "/1
  b/1 -> Gain3/1, Gain11/1
  Gain1/1 -> Sum/3
  a/1 -> Gain2/1, Sum/1

== system afe_dq_ttype/afe_dq_mod1/AFE_control/afe_control/instantaneus_power/abc2alphabeta  ==
  a : Inport
  b : Inport  Port=2
  c : Inport  Port=3
  Gain1 : Gain  Gain=-1/2
  Gain11 : Gain  Gain=-1/2
  Gain2 : Gain  Gain=0
  Gain3 : Gain  Gain=sqrt(3)/2
  Gain4 : Gain  Gain=-sqrt(3)/2
  Gain8 : Gain  Gain=2/3
  Gain9 : Gain  Gain=2/3
  Sum : Sum  Inputs=+++
  Sum1 : Sum  Inputs=+++
  "alpha " : Outport  VectorParamsAs1DForOutWhenUnconnected=off
  "beta " : Outport  Port=2  VectorParamsAs1DForOutWhenUnconnected=off
  wires:
  a/1 -> Sum/1, Gain2/1
  Gain2/1 -> Sum1/1
  Gain9/1 -> "beta "/1
  Gain11/1 -> Sum/2
  c/1 -> Gain1/1, Gain4/1
  Sum/1 -> Gain8/1
  Sum1/1 -> Gain9/1
  Gain1/1 -> Sum/3
  Gain3/1 -> Sum1/2
  Gain4/1 -> Sum1/3
  Gain8/1 -> "alpha "/1
  b/1 -> Gain11/1, Gain3/1

== system afe_dq_ttype/afe_dq_mod1/AFE_control/afe_control/instantaneus_power/moving_avarage_p ==
  in : Inport
  Gain : Gain  Gain=param.afe.ctrl.rms.n1-1
  Gain1 : Gain  Gain=1/param.afe.ctrl.rms.n1
  Sum : Sum  Inputs=|++
  Unit Delay : UnitDelay  SampleTime=-1
  out : Outport  VectorParamsAs1DForOutWhenUnconnected=off
  wires:
  Gain/1 -> Sum/2
  Gain1/1 -> out/1, Unit Delay/1
  in/1 -> Sum/1
  Unit Delay/1 -> Gain/1
  Sum/1 -> Gain1/1

== system afe_dq_ttype/afe_dq_mod1/AFE_control/afe_control/instantaneus_power/moving_avarage_q ==
  in : Inport
  Gain : Gain  Gain=param.afe.ctrl.rms.n1-1
  Gain1 : Gain  Gain=1/param.afe.ctrl.rms.n1
  Sum : Sum  Inputs=|++
  Unit Delay : UnitDelay  SampleTime=-1
  out : Outport  VectorParamsAs1DForOutWhenUnconnected=off
  wires:
  Sum/1 -> Gain1/1
  Unit Delay/1 -> Gain/1
  in/1 -> Sum/1
  Gain1/1 -> Unit Delay/1, out/1
  Gain/1 -> Sum/2

== system afe_dq_ttype/afe_dq_mod1/AFE_control/afe_control/instantaneus_power/rms ==
  In1 : Inport
  Gain : Gain  Gain=param.afe.ctrl.rms.n10-1
  Gain1 : Gain  Gain=1/param.afe.ctrl.rms.n10
  Math Function : Math  Operator=magnitude^2  SignedPower=on
  Sqrt : Sqrt
  Sum : Sum  Inputs=|++
  Unit Delay : UnitDelay  SampleTime=-1
  Out1 : Outport  VectorParamsAs1DForOutWhenUnconnected=off
  wires:
  In1/1 -> Math Function/1
  Sum/1 -> Gain1/1
  Gain1/1 -> Sqrt/1, Unit Delay/1
  Unit Delay/1 -> Gain/1
  Math Function/1 -> Sum/1
  Sqrt/1 -> Out1/1
  Gain/1 -> Sum/2

== system afe_dq_ttype/afe_dq_mod1/AFE_control/afe_control/instantaneus_power/rms1 ==
  In1 : Inport
  Gain : Gain  Gain=param.afe.ctrl.rms.n10-1
  Gain1 : Gain  Gain=1/param.afe.ctrl.rms.n10
  Math Function : Math  Operator=magnitude^2  SignedPower=on
  Sqrt : Sqrt
  Sum : Sum  Inputs=|++
  Unit Delay : UnitDelay  SampleTime=-1
  Out1 : Outport  VectorParamsAs1DForOutWhenUnconnected=off
  wires:
  Gain/1 -> Sum/2
  Sqrt/1 -> Out1/1
  Math Function/1 -> Sum/1
  Unit Delay/1 -> Gain/1
  Gain1/1 -> Unit Delay/1, Sqrt/1
  Sum/1 -> Gain1/1
  In1/1 -> Math Function/1

== system afe_dq_ttype/afe_dq_mod1/AFE_control/afe_control/instantaneus_power/rms2 ==
  In1 : Inport
  Gain : Gain  Gain=param.afe.ctrl.rms.n10-1
  Gain1 : Gain  Gain=1/param.afe.ctrl.rms.n10
  Math Function : Math  Operator=magnitude^2  SignedPower=on
  Sqrt : Sqrt
  Sum : Sum  Inputs=|++
  Unit Delay : UnitDelay  SampleTime=-1
  Out1 : Outport  VectorParamsAs1DForOutWhenUnconnected=off
  wires:
  In1/1 -> Math Function/1
  Sum/1 -> Gain1/1
  Gain1/1 -> Sqrt/1, Unit Delay/1
  Unit Delay/1 -> Gain/1
  Math Function/1 -> Sum/1
  Sqrt/1 -> Out1/1
  Gain/1 -> Sum/2

== system afe_dq_ttype/afe_dq_mod1/AFE_control/afe_control/instantaneus_power/rms3 ==
  In1 : Inport
  Gain : Gain  Gain=param.afe.ctrl.rms.n10-1
  Gain1 : Gain  Gain=1/param.afe.ctrl.rms.n10
  Math Function : Math  Operator=magnitude^2  SignedPower=on
  Sqrt : Sqrt
  Sum : Sum  Inputs=|++
  Unit Delay : UnitDelay  SampleTime=-1
  Out1 : Outport  VectorParamsAs1DForOutWhenUnconnected=off
  wires:
  Gain/1 -> Sum/2
  Sqrt/1 -> Out1/1
  Math Function/1 -> Sum/1
  Unit Delay/1 -> Gain/1
  Gain1/1 -> Unit Delay/1, Sqrt/1
  Sum/1 -> Gain1/1
  In1/1 -> Math Function/1

== system afe_dq_ttype/afe_dq_mod1/AFE_control/afe_control/instantaneus_power/rms4 ==
  In1 : Inport
  Gain : Gain  Gain=param.afe.ctrl.rms.n10-1
  Gain1 : Gain  Gain=1/param.afe.ctrl.rms.n10
  Math Function : Math  Operator=magnitude^2  SignedPower=on
  Sqrt : Sqrt
  Sum : Sum  Inputs=|++
  Unit Delay : UnitDelay  SampleTime=-1
  Out1 : Outport  VectorParamsAs1DForOutWhenUnconnected=off
  wires:
  In1/1 -> Math Function/1
  Sum/1 -> Gain1/1
  Gain1/1 -> Sqrt/1, Unit Delay/1
  Unit Delay/1 -> Gain/1
  Math Function/1 -> Sum/1
  Sqrt/1 -> Out1/1
  Gain/1 -> Sum/2

== system afe_dq_ttype/afe_dq_mod1/AFE_control/afe_control/instantaneus_power/rms5 ==
  In1 : Inport
  Gain : Gain  Gain=param.afe.ctrl.rms.n10-1
  Gain1 : Gain  Gain=1/param.afe.ctrl.rms.n10
  Math Function : Math  Operator=magnitude^2  SignedPower=on
  Sqrt : Sqrt
  Sum : Sum  Inputs=|++
  Unit Delay : UnitDelay  SampleTime=-1
  Out1 : Outport  VectorParamsAs1DForOutWhenUnconnected=off
  wires:
  Gain/1 -> Sum/2
  Sqrt/1 -> Out1/1
  Math Function/1 -> Sum/1
  Unit Delay/1 -> Gain/1
  Gain1/1 -> Unit Delay/1, Sqrt/1
  Sum/1 -> Gain1/1
  In1/1 -> Math Function/1

== system afe_dq_ttype/afe_dq_mod1/afe/deadtime_generator_for_ttype/dead_time_generator_cmos_simulink_phu/dead_time_leg_generator_1 ==
  cmd_in_QA : Inport
  cmd_in_QB : Inport  Port=2
  MATLAB Function : MATLAB Function  TreatAsAtomicUnit=on
  MATLAB Function1 : MATLAB Function  TreatAsAtomicUnit=on
  MATLAB Function2 : MATLAB Function  TreatAsAtomicUnit=on
  MATLAB Function3 : MATLAB Function  TreatAsAtomicUnit=on
  MATLAB Function4 : MATLAB Function  TreatAsAtomicUnit=on
  MATLAB Function5 : MATLAB Function  TreatAsAtomicUnit=on
  MATLAB Function6 : MATLAB Function  TreatAsAtomicUnit=on
  MATLAB Function7 : MATLAB Function  TreatAsAtomicUnit=on
  MATLAB Function8 : MATLAB Function  TreatAsAtomicUnit=on
  MATLAB Function9 : MATLAB Function  TreatAsAtomicUnit=on
  Transfer Fcn : TransferFcn  Denominator=[sqrt(2)*deadtime 1]
  Transfer Fcn1 : TransferFcn  Denominator=[sqrt(2)*deadtime 1]
  cmd_out_QA : Outport
  cmd_out_QB : Outport  Port=2
  wires:
  MATLAB Function8/1(y) -> MATLAB Function5/2(u2)
  MATLAB Function7/1(y) -> Transfer Fcn1/1, MATLAB Function9/2(u2)
  MATLAB Function3/1(y) -> MATLAB Function1/2(u2)
  MATLAB Function2/1(y) -> Transfer Fcn/1, MATLAB Function4/1(u1)
  MATLAB Function/1(y) -> MATLAB Function1/1(u1), MATLAB Function2/1(u)
  MATLAB Function9/1(y) -> cmd_out_QB/1
  MATLAB Function4/1(y) -> cmd_out_QA/1
  MATLAB Function6/1(y) -> MATLAB Function5/1(u1), MATLAB Function7/1(u)
  cmd_in_QA/1 -> MATLAB Function/1(u)
  MATLAB Function5/1(y) -> MATLAB Function4/2(u2)
  MATLAB Function1/1(y) -> MATLAB Function9/1(u1)
  cmd_in_QB/1 -> MATLAB Function6/1(u)
  Transfer Fcn1/1 -> MATLAB Function8/1(u)
  Transfer Fcn/1 -> MATLAB Function3/1(u)
